simulink model "InductionHeating_bb_4"  (R2026b)
settings: Solver=FixedStepDiscrete  StopTime=0.008
PostLoadFcn:
  | Ts = 1e-6;Ts_fpga=10e-9;   R=3; Capa=300e-9;L=100e-6;Pejo_factor=1;
InitFcn:
  | Ts = 1e-6;Ts_fpga=10e-9;   R=3; Capa=300e-9;L=100e-6;Pejo_factor=1;
undefined symbols (not defined in the file or in its folder): DiscIntNeverNeededParam, ee_sli_rtmsupport, gcbh, isSetWhenUndefinedState, MATESOCwDio
libraries: fl_lib x67, nesl_utility x40, hdlsllib x32, simulink x15, eeGeneralControl x9, ee_lib x3
(part 1 of 7)
settings Model: DataTypeOverride=Off  ModifiedByFormat=sss  Creator=The MathWorks, Inc.  LastModifiedBy=sss
settings OptimizationCC: BlockReduction=off  ConditionallyExecuteInputs=off  DefaultParameterBehavior=Inlined  InheritOutputTypeSmallerThanSingle=on  ReuseModelBlockBuffer=off
settings DebuggingCC: AlgebraicLoopMsg=error  ParameterPrecisionLossMsg=none  SingleTaskRateTransMsg=error  SubsystemReferenceDiagnosticForUnitTest=warning
settings HardwareCC: ProdEndianess=Unspecified  ProdEqTarget=off  ProdHWDeviceType=ASIC/FPGA->ASIC/FPGA  ProdIntDivRoundTo=Undefined  ProdLargestAtomicFloat=None  TargetEndianess=LittleEndian  TargetHWDeviceType=Custom Processor->MATLAB Host Computer  TargetIntDivRoundTo=Zero  TargetLongLongMode=on
settings RTWCC: DLArmComputeVersion=19.05
settings SimscapeCC: SimscapeUseEnergyAccounting=off

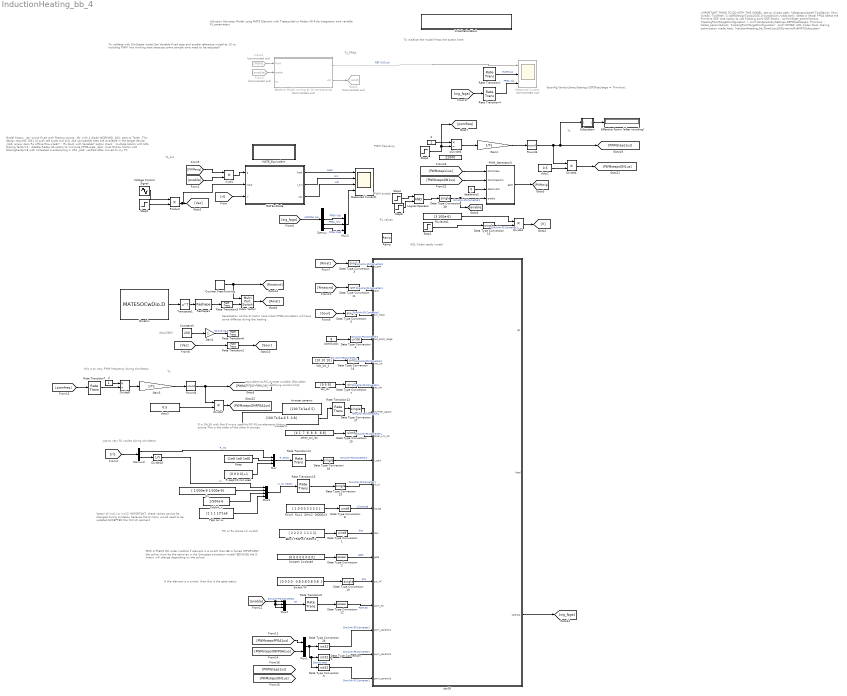
== system InductionHeating_bb_4 ==
  note: Model history
      | _aa: circuit fixed with floating source
      | _bb: with 4 diode WORKING
      | _bb1: sent to Tarek: This design requires 1041 of such cell types but only 464 compatible sites are available in the target device.
      | _bb2: erreur dans RL offline Rsw+1e6!!!
      | : RL block with VariableY option check
      | : multiple blocks with HDL sharing factor=4
      | : disable Radau IIA option to minimize FPGA area
      | _bb3: most RLCsw blocks with SharingFactor=8
      | with increased oversampling = 254
      | _bb4: verified after moved to my PC
  note: I MPORTANT THING TO DO WITH THIS MODEL:
      |
      | set-up Vivado path: hdlsetuptoolpath('ToolName','Xilinx Vivado','ToolPath','C:\AMDDesignTools\2026.1\Vivado\bin\vivado.bat');
      |
      | Select a Versal FPGA
      |
      | Select the Primitive DSP slice option to use Floating point DSP blocks.:
      | conf=hdlget_param(bdroot, 'FloatingPointTargetConfiguration' );
      | conf.VendorLibrarySettings.DSPSliceUsage= 'Primitive' ;
      | hdlset_param(bdroot, 'FloatingPointTargetConfiguration' ,conf)
      |
      | NOTES:
      | HDL Coder block sharing optimization made here: 'InductionHeating_bb_Tarek/soc16/DynamicMultMAT/Subsystem'
  note: Vdc=200V
  note: equivalent to RC inverter snubber
      | [Rsnubber Ts/Csnubber  non-rectifying current limit]
  note: D is 16x16
      | with first 8 in-out used for RC-RL-sw elements History source
      | This is the order of the other 8 sources
  note: this is to vary PWM frequency during simulation
  note: If the element is a switch, then this is the gate status
  note: just to vary RL vaules during simulation
  note: RC or RL choice (or switch)
  note: Vector of inv(L) or inv(C)
      | IMPORTANT: these values cannot be changed during simlation
      | because the D marix would need to be updated
      | EXCEPTED the first LC element
  note: IRK5 is PLECS 5th order method
      | if element is a switch then BE is forced
      | IMPORTANT: the solver must be the same as in the Simscape extraction model!
      | BECAUSE the D matrix will change depending on the solver!
  note: Ts
  note: Induction Stovetop Model using MATE Element
      | with Trapezoidal or Radau IIA Rule Integration
      | and variable RL parameters
  note: Serialisation od the D matrix here
      | Initial FPGA simulation will have some diffence during the loading
  note: HDL Coder ready model
  note: Ts
  note: Ts_FPGA
  note: To validate with SimScape model
      | Set Variable fixed step and enable reference model
      | at 10 ns including PWM
      | (not working here because some sample time need to be adjusted)
  note: Ts_1us
  note: RL values
  note: PWM frequency
  note: PWM enable
  note: fpconfig.VendorLibrarySettings.DSPSliceUsage = 'Primitive';
  note: To initialize the model
      |
      | Press the button here
  0=open 1=closed : Constant  Value=[0 0 0 0 0 0 0 0]  OutDataTypeStr=boolean  SampleTime=Ts
  1 : Constant  Value=22000  SampleTime=Ts
  3 : Constant  SampleTime=Ts
  4 : Constant  SampleTime=Ts
  BE=1 TRAP=2 IRK5=3 _ : Constant  Value="[ 2 2 2 2  1 1 1 1]"  OutDataTypeStr=single  SampleTime=Ts
  Baseline Model running at 10 nanoseconds : Subsystem  Commented=on
  Cdclink_x : Constant  Value=1/500e-6  OutDataTypeStr=single  SampleTime=Ts
  Constant : Constant  Value="[100 Ts/1e-6 5  0.8]"
  Constant3 : Constant  Value=200  SampleTime=Ts
  Counter Free-Running : hdlsllib/Sources/Counter Free-Running  NumBits=8  tsamp=-1
  Cx : Constant  Value=[ 1/300e-9 1/300e-9]  OutDataTypeStr=single  SampleTime=Ts
  Data Type Conversion{1,4,7..8,11,15..16} (7 alike) : DataTypeConversion  OutDataTypeStr=uint8  RndMeth=Nearest  SaturateOnIntegerOverflow=off
  Data Type Conversion{3,5,10,13,18..19,37..38} (8 alike) : DataTypeConversion  OutDataTypeStr=single  RndMeth=Nearest  SaturateOnIntegerOverflow=off
  Data Type Conversion12 : DataTypeConversion  OutDataTypeStr=boolean  RndMeth=Nearest  SaturateOnIntegerOverflow=off
  Data Type Conversion2 : DataTypeConversion  OutDataTypeStr=boolean  RndMeth=Nearest  SaturateOnIntegerOverflow=off
  Data Type Conversion28 : DataTypeConversion  OutDataTypeStr=int32  RndMeth=Nearest  SaturateOnIntegerOverflow=off
  Data Type Conversion6 : DataTypeConversion  OutDataTypeStr=int32  RndMeth=Nearest  SaturateOnIntegerOverflow=off
  Data Type Conversion9 : DataTypeConversion  OutDataTypeStr=int32  RndMeth=Nearest  SaturateOnIntegerOverflow=off
  Demux : Demux  Outputs=5
  Demux3 : Demux  Outputs=[1 1]
  Divide1 : Product
  Divide10 : Product  Inputs=/
  Divide4 : Product
  Divide6 : Product  Inputs=*/
  Divide7 : Product
  Divide8 : Product  Inputs=*/
  Dmatrix : Constant  Value=MATESOCwDio.D
  Effective Fpwm (after rounding) : Display
      settings: Format=bank
  From2 : From  Commented=on  GotoTag=enable
  From3 : From  Commented=on  GotoTag=PWM
  Gain1 : Gain  Gain=1/Ts
  Gain2 : Gain
  Gain3 : Gain  Gain=1/Ts
  Goto1 : Goto  Commented=on  GotoTag=vdcref
  Index Vector : MultiPortSwitch  DataPortOrder=Zero-based contiguous  Inputs=1  zeroidx=on  SaturateOnIntegerOverflow=off  InputSameDT=off
  InitializationBlock : Subsystem  AncestorBlock=simetranss/Usefulls/InitializationBlock  mask(Model Functions){InitVar=Ts = 1e-6;Ts_fpga=10e-9;   R=3; Capa=300e-9;L=100e-6;Pejo_factor=1;, InitFile=, prel=off, posl=on, inif=on}
      mask prompts: InitVar "Initialisation variables"; InitFile "Initialisation file (.m or .p)"; prel "Preload Function"; posl "PostLoad Function"; inif "InitFcn"
      mask init:
      | InitAll=[InitVar 10 InitFile];
      | if prel==1
      | 	set_param(bdroot, 'PreLoadFcn', InitAll);
      | else
      | 	set_param(bdroot, 'PreLoadFcn', '');
      | end
      | if inif==1
      | 	set_param(bdroot, 'InitFcn', InitAll);
      | else
      | 	set_param(bdroot, 'InitFcn', '');
      | end
      | 
      | if posl==1
      | 	set_param(bdroot, 'PostLoadFcn', InitAll);
      | else
      | 	set_param(bdroot, 'PostLoadFcn', '');
      | end
      | 
      | 
      | 
      | pos = get_param(gcb, 'Position');
      | width = pos(3) - pos(1); height = pos(4) - pos(2);
      mask DialogControl openfile Prompt: Open Initialisation file
      mask DialogControl openfile Callback:
      | ff1=get_param(gcb,'InitFile');
      | ff=replace(ff1,';','');
      | ff=replace(ff,'.m','');
      | ff=replace(ff,'.p','');
      | 
      | if ~isempty(strfind(ff1,'.p'))
      |     warning('p-file cannot be edited')
      | end
      | 
      | open(ff);
      mask Display:
      | text(5, height*0.5, [ ...
      |   ...
      | '- Initialisation: '  get_param(bdroot, 'InitFcn')  ...
      | ], ...
      | 'horizontalAlignment', 'left', 'verticalAlignment', 'middle') ;
  Inverter params : Constant  Value=[100 Ts/1e-6 5]
  Logical Operator : Logic  AllPortsSameDT=off  OutDataTypeStr=boolean
  MATE_Equivalent : Subsystem  mask(MATE object){MATEin='MATE', MATERT='MATERT', MATESOCvar='MATESOCwDio', subsys='InductionHeating_bb_4/MATEwDiode', discmeth=Trapezoidal, Tsx=Ts}
      mask prompts: MATEin "General MATE data structure name"; MATERT "MATE S-function parameter"; MATESOCvar "MATE-SoC output variable name"; subsys "Reference subsystem for MATE"; discmeth "Discretization"; Tsx "Sample time (s)"
      mask TypeOptions discmeth: Backward Euler | Trapezoidal |  5th order accurate fully-implicit three-stage Runge-Kutta formula (Radau IIA)
      mask DialogControl Control2 Prompt: Generate MATE equations
      mask DialogControl Control2 Callback:
      | block=gcb;
      | maskObj = Simulink.Mask.get(block); % get mask handle
      | Ts = get_param(block, 'value@Tsx'); % retrieve value for Vrated
      | sub = get_param(block, 'value@subsys'); % retrieve value for Vmin_p
      | dd = get_param(block, 'value@discmeth'); % retrieve value for Vmin_p
      | mm = get_param(block, 'value@MATEin'); % retrieve value for Vmin_p
      | mrt = get_param(block, 'value@MATERT'); % retrieve value for Vmin_p
      | msoc = get_param(block, 'value@MATESOCvar'); % retrieve value for Vmin_p
      | if dd==3
      |     dd=5;
      | end
      | %Tss=get_param(block,'Ts')
      | [MATEx, MATERTx]= MakeMate2(sub , dd, Ts);
      | %MATEin='MATE';
      | assignin("base",mm,MATEx);
      | assignin("base",mrt,MATERTx);
      | [MATESOCx]=MateConvertForFPGA(MATEx,2);  % don;t forget option 2
      | assignin("base",msoc,MATESOCx);
  MATEwDiode : Subsystem
  Measured Current : Scope  Commented=on  NumInputPorts=3
      settings: ActiveDisplayYMinimum=-142.71321105957031  ActiveDisplayYMaximum=758.74385070800781
  Measured Current1 : Scope  NumInputPorts=4
      settings: ActiveDisplayYMinimum=-62.985793783247914  ActiveDisplayYMaximum=66.216303930478091
  Mux : Mux  Inputs=3
  Mux1 : Mux  Inputs=2
  Mux2 : Mux  Inputs=3
  Mux3 : Mux  Inputs=3
  Mux5 : Mux
  PWM_Generator3 : Subsystem
      mask Display: disp(' PWM \n Generator ')
  Pejo sw Lx : Constant  Value=[1 1 1 1]*1e6  OutDataTypeStr=single  SampleTime=Ts
  Product : Product
  R pejo=0 not used : Constant  Value=[0 0 0 0]+1  OutDataTypeStr=single  SampleTime=Ts
  RC=0  RL=1  SW=2  DIODE=3 : Constant  Value=[ 1 0 0 0 3 3 3 3 ]  OutDataTypeStr=single  SampleTime=Ts
  RLvlaues1 : Constant  Value=[3 100e-6]  OutDataTypeStr=single  SampleTime=Ts
  Ramp : simulink/Sources/Ramp  slope=-0.1*1000  start=0.004  InitialOutput=1
  Rate Transition1 : RateTransition  Integrity=off
  Rate Transition{5,7,13..15} (5 alike) : RateTransition  Integrity=off  OutPortSampleTime=Ts
  Rate Transition2 : RateTransition  OutPortSampleTime=1e-06
  Rate Transition3 : RateTransition  OutPortSampleTime=1e-06
  Rate Transition4 : RateTransition  Integrity=off
  Rate Transition6 : RateTransition  OutPortSampleTime=1e-06
  Rcap : Constant  Value=[1e8 1e8 1e8]  OutDataTypeStr=single  SampleTime=Ts
  Reshape1 : Reshape
  Round3 : Rounding  Operator=round
  Round4 : Rounding  Operator=round
  Step1 : Step  Time=0.004  InitialValue=1  FinalValue=0.9  SampleTime=Ts
  Step2 : Step  Time=0.002  SampleTime=Ts
  Step3 : Step  Time=0.001  SampleTime=Ts
  Step4 : Step  Time=0.003  InitialValue=25000  FinalValue=22000  SampleTime=Ts
  Step6 : Step  Time=0.005  InitialValue=1  FinalValue=0  SampleTime=Ts
  Subsystem : Subsystem
  Switch VF : Constant  Value="[0 0 0 0   0.8 0.8 0.8 0.8  ]"  OutDataTypeStr=single  SampleTime=Ts
  Transpose1 : Math  Operator=transpose
  UserOutidx : Constant  Value=9  SampleTime=Ts
  Vdc_idx_1 : Constant  Value=[10 10 10]  SampleTime=Ts
  Voltage Control Signal : Sin  Amplitude=220  Frequency=500 * 2 *pi  SampleTime=Ts
  deadtime2 : Constant  Value=0  SampleTime=Ts
  duty2 : Constant  Value=0.5  SampleTime=Ts
  duty3 : Constant  Value=0.5  SampleTime=Ts
  iac_idx : Constant  Value=[9 9 9]  SampleTime=Ts
  mult1 : Product
  other_src_idx : Constant  Value="[4 1  7  8  8  8   8 8]"  SampleTime=Ts
  soc16 : Subsystem  TreatAsAtomicUnit=on
  wires:
  Rate Transition1/1 -> Measured Current/2  "MATE 1us"
  Baseline Model running at 10 nanoseconds/1(i) -> Measured Current/1  "REF (0.01 us)"
  From2/1 -> Baseline Model running at 10 nanoseconds/2(enable)
  Baseline Model running at 10 nanoseconds/2(vdc) -> Goto1/1
  From3/1 -> Baseline Model running at 10 nanoseconds/1(PWM)
  Rate Transition4/1 -> Measured Current/3  "FPGA 1us"
  [Rmat] -> Data Type Conversion3/1
  Counter Free-Running/1 -> Index Vector/1, [Rmatcnt]
  Dmatrix/1 -> Transpose1/1
  Transpose1/1 -> Reshape1/1
  Reshape1/1 -> Rate Transition3/1
  Rate Transition3/1 -> Index Vector/2
  Gain2/1 -> Rate Transition6/1  "Source input"
  [Rmatcnt] -> Data Type Conversion11/1
  Index Vector/1 -> [Rmat]
  [Sour] -> Data Type Conversion5/1
  Constant3/1 -> Gain2/1
  [PWMstepsFPGA1us] -> Mux1/1
  [PWMstepsONFPGA1us] -> Mux1/2
  Mux1/1 -> Data Type Conversion9/1, Data Type Conversion6/1, Data Type Conversion28/1  "Source input"
  Data Type Conversion28/1 -> soc16/16(pwm_params1)  "Simulink-PS Converter1"
  Data Type Conversion37/1 -> soc16/7(inverter_param)  "Simulink-PS Converter1"
  [PWMstepsON1us] -> PWM_Generator3/2(PWMstepsON)
  [PWMsteps1us] -> PWM_Generator3/1(PWMsteps)
  deadtime2/1 -> PWM_Generator3/3(deatime(s))
  duty2/1 -> Divide4/2
  Divide4/1 -> [PWMstepsON1us]
  Round3/1 -> Divide4/1, Subsystem/1(In1), [PWMsteps1us]
  Divide6/1 -> Gain1/1
  Gain1/1 -> Round3/1
  3/1 -> Divide6/1
  Data Type Conversion38/1 -> [enable], PWM_Generator3/4(enable)  "Simulink-PS Converter1"
  PWM_Generator3/1(gate) -> [PWMavg]
  Data Type Conversion3/1 -> soc16/1(d_port)  "Simulink-PS Converter1"
  Data Type Conversion11/1 -> soc16/2(dcnt)  "Simulink-PS Converter1"
  Data Type Conversion5/1 -> soc16/3(src_input)  "Simulink-PS Converter1"
  4/1 -> Divide8/1
  Divide8/1 -> Gain3/1
  Gain3/1 -> Round4/1
  duty3/1 -> Divide7/2
  Rate Transition7/1 -> Divide8/2
  Round4/1 -> [PWMstepsFPGA1us], Divide7/1
  Divide7/1 -> [PWMstepsONFPGA1us]
  Rate Transition13/1 -> Data Type Conversion37/1
  [sig_fpga] -> Rate Transition4/1
  [pwmfreq] -> Rate Transition7/1
  other_src_idx/1 -> Data Type Conversion15/1
  iac_idx/1 -> Data Type Conversion7/1
  UserOutidx/1 -> Data Type Conversion4/1
  Data Type Conversion4/1 -> soc16/4(out_start_range)  "Simulink-PS Converter1"
  Vdc_idx_1/1 -> Data Type Conversion16/1  "Simulink-PSConverter1"
  Data Type Conversion7/1 -> soc16/6(iac_idx)  "Simulink-PS Converter1"
  Data Type Conversion16/1 -> soc16/5(vdc_idx)  "Simulink-PS Converter1"
  Data Type Conversion15/1 -> soc16/8(other_src_idx)  "Simulink-PS Converter1"
  Mux5/1 -> Rate Transition15/1  "Lx_Cx vector"
  Demux3/2 -> Divide10/1
  Mux/1 -> Rate Transition14/1  "R vector"
  Data Type Conversion18/1 -> soc16/9(r_port)  "Simulink-PS Converter1"
  Data Type Conversion19/1 -> soc16/10(lx_cx)  "Simulink-PS Converter1"
  Rate Transition14/1 -> Data Type Conversion18/1
  Rate Transition15/1 -> Data Type Conversion19/1
  Data Type Conversion8/1 -> soc16/11(lctype)  "LCswtype"
  Data Type Conversion1/1 -> soc16/12(disc)  "disc"
  Data Type Conversion2/1 -> soc16/13(gate)  "gate"
  RC=0  RL=1  SW=2  DIODE=3/1 -> Data Type Conversion8/1
  0=open 1=closed/1 -> Data Type Conversion2/1
  BE=1 TRAP=2 IRK5=3 _/1 -> Data Type Conversion1/1
  Rate Transition5/1 -> Data Type Conversion12/1
  Data Type Conversion12/1 -> soc16/15(pwm_en)  "PWM en"
  Data Type Conversion6/1 -> soc16/17(pwm_params2)  "Simulink-PS Converter1"
  Data Type Conversion9/1 -> soc16/18(pwm_params3)  "Simulink-PS Converter1"
  [enable] -> Mux2/3, Mux2/2, Mux2/1  "Simulink-PS Converter1"
  Mux2/1 -> Rate Transition5/1  "en"
  mult1/1 -> MATEwDiode/1(g)
  [PWMavg] -> mult1/1
  [enable] -> mult1/2
  MATEwDiode/3(vdc) -> Measured Current1/3  "Vdc"
  MATEwDiode/1(iload) -> Measured Current1/1  "Iload"
  MATEwDiode/2(i_src) -> Measured Current1/2  "Isrc"
  Subsystem/1(Out1) -> Effective Fpwm (after rounding)/1
  Switch VF/1 -> Data Type Conversion10/1
  Data Type Conversion10/1 -> soc16/14(sw_VF)  "disc"
  Step4/1 -> [pwmfreq], Divide6/2
  [Vac] -> Rate Transition2/1
  Rate Transition2/1 -> [Sour]
  Demux3/1 -> Mux/1  "R_ind"
  Rcap/1 -> Mux/2
  R pejo=0 not used/1 -> Mux/3
  Divide10/1 -> Mux5/1  "Lx"
  Cx/1 -> Mux5/2
  Cdclink_x/1 -> Mux5/3
  Pejo sw Lx/1 -> Mux5/4
  soc16/3(userout) -> [sig_fpga]
  Divide1/1 -> [rl]
  Data Type Conversion13/1 -> Divide1/2  "Simulink-PS Converter1"
  RLvlaues1/1 -> Divide1/1
  [rl] -> MATEwDiode/3(rl)
  [rl] -> Demux3/1
  Step2/1 -> Logical Operator/1
  Step6/1 -> Logical Operator/2
  Logical Operator/1 -> Data Type Conversion38/1
  Step3/1 -> Product/2
  Voltage Control Signal/1 -> Product/1
  Product/1 -> MATEwDiode/2(Input), [Vac]
  Constant/1 -> Rate Transition13/1
  [sig_fpga] -> Demux/1  "vdcFPGA 1us"
  Demux/5 -> Mux3/3  "FPGA Iload"
  Mux3/1 -> Measured Current1/4
  Demux/4 -> Mux3/2  "FPGA_Isrc"
  Demux/3 -> Mux3/1  "FPGA Vdc"
  Step1/1 -> Data Type Conversion13/1

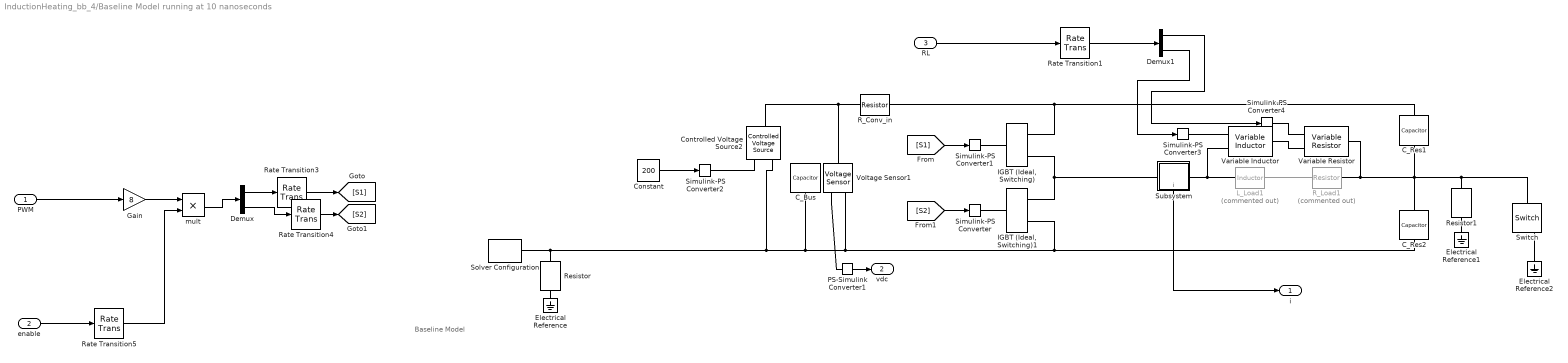
== system InductionHeating_bb_4/Baseline Model running at 10 nanoseconds ==
  note: Baseline Model
  PWM : Inport
  enable : Inport  Port=2
  RL : Inport  Port=3
  C_Bus : fl_lib/Electrical/Electrical Elements/Capacitor  c=5e-5 F  r=0 Ohm  g=0 1/Ohm  i_specify=off  i_priority=None  i=0 A  i_nominal_specify=off  i_nominal_value=1  i_nominal_unit=A  v_specify=off  v_priority=None  v=0 V  v_nominal_specify=off  v_nominal_value=1  v_nominal_unit=V  vc_specify=off  vc_priority=High  vc=0 V  vc_nominal_specify=off  vc_nominal_value=1  vc_nominal_unit=V
      settings: AttributesFormatString=%<c> %<c_unit>
  C_Res1 : fl_lib/Electrical/Electrical Elements/Capacitor  c=300e-9 F  r=0 Ohm  g=0 1/Ohm  i_specify=off  i_priority=None  i=0 A  i_nominal_specify=off  i_nominal_value=1  i_nominal_unit=A  v_specify=off  v_priority=None  v=0 V  v_nominal_specify=off  v_nominal_value=1  v_nominal_unit=V  vc_specify=off  vc_priority=High  vc=0 V  vc_nominal_specify=off  vc_nominal_value=1  vc_nominal_unit=V
      settings: AttributesFormatString=%<c> %<c_unit>
  C_Res2 : fl_lib/Electrical/Electrical Elements/Capacitor  c=300e-9 F  r=0 Ohm  g=0 1/Ohm  i_specify=off  i_priority=None  i=0 A  i_nominal_specify=off  i_nominal_value=1  i_nominal_unit=A  v_specify=off  v_priority=None  v=0 V  v_nominal_specify=off  v_nominal_value=1  v_nominal_unit=V  vc_specify=off  vc_priority=High  vc=0 V  vc_nominal_specify=off  vc_nominal_value=1  vc_nominal_unit=V
      settings: AttributesFormatString=%<c> %<c_unit>
  Constant : Constant  Value=200
  Controlled Voltage Source2 : fl_lib/Electrical/Electrical Sources/Controlled Voltage Source
  Demux : Demux  Outputs=2
  Demux1 : Demux  Outputs=2
  Electrical Reference : fl_lib/Electrical/Electrical Elements/Electrical Reference
  Electrical Reference1 : fl_lib/Electrical/Electrical Elements/Electrical Reference
  Electrical Reference2 : fl_lib/Electrical/Electrical Elements/Electrical Reference
  Gain : Gain  Gain=8
  "IGBT (Ideal, Switching)" : ee_lib/Semiconductors & Converters/IGBT (Ideal, Switching)  port_option=ee.enum.controlport.ps  Vf=0.8 V  Ron=0.001 Ohm  Goff=1e-8 1/Ohm  Vth=6 V  diode_param=2  diode_Vf=0.8 V  diode_Ron=0.001 Ohm  diode_Goff=1e-8 1/Ohm  diode_C=50e-9 F  diode_iRM=-235 A  diode_iF=300 A  diode_idot=-50 A/us  diode_trr_param=1  diode_trr_factor=3  diode_trr=15 us  diode_Qrr=1500 s*uA  ice_specify=off  ice_priority=None  ice=0 A  ice_nominal_specify=off  ice_nominal_value=1  ice_nominal_unit=A  vce_specify=off  vce_priority=None  vce=0 V  vce_nominal_specify=off  vce_nominal_value=1  vce_nominal_unit=V  vge_specify=off  vge_priority=None  vge=0 V  vge_nominal_specify=off  vge_nominal_value=1  vge_nominal_unit=V  thermal_loss_option=ee.enum.converters.thermalLossOption.constantvalues  Von_data=[0, .1, .6, .8, 1, 1.3, 1.6, 2, 2.4; 0, .1, .7, 1, 1.2, 1.5, 1.9, 2.4, 2.8] V  Tj=[298.15, 398.15] K  Iout_data=[0, .1, 1, 5, 10, 20, 40, 70, 100] A  Eon_data=[0, .0024, .024, .12, .2, .48, 1.04, 2.16, 3.24; 0, .003, .03, .15, .25, .6, 1.3, 2.7, 4.05] * 1e-3 J  Eoff_data=[0, .0007, .0066, .033, .066, .17, .33, .83, 1.5; 0, .001, .01, .05, .1, .25, .5, 1.2, 2.2] * 1e-3 J  Eon_data_3D=[zeros(2, 9, 3)] J  Eoff_data_3D=[zeros(2, 9, 3)] J  Tj_loss=[298.15, 398.15] K  Iout_data_loss=[0, .1, 1, 5, 10, 20, 40, 70, 100] A  tabulateWithVce=false  Vce_loss=[0, 150, 300] V  Eon_scalar=22.86e-3 J  Eoff_scalar=17.14e-3 J  Voff=300 V  Iout_scalar=600 A  useCurrentFromPreviousCycle=false  useVoltageFromPreviousCycle=false  diodeModelType=ee.enum.converters.diodeModelType.pwl  diodeTableType=ee.enum.diode.tableType.IfMat  diode_ReverseIVType=ee.enum.diode.diodeReverseIV.constant  diode_IfMat=[.07, .12, .19, 1.75, 4.24, 7.32, 11.2; .16, .3, .72, 2.14, 4.02, 6.35, 9.12] A  diode_VfMat=[.9, 1.15, 1.25, 1.5, 1.75, 2.17, 2.6, 2.85; .58, .68, .75, 1.1, 1.38, 1.77, 2.27, 2.7] V  diode_TjVec=[25, 125] degC  diode_VfVec=[.5, .7, .9, 1.3, 1.7, 2.1, 2.5] V  diode_IfVec=[.1, .2, .5, 1, 2, 4, 7, 10] A  diode_IrMat=[1e-06, 2e-06, 5e-06, 1e-05, 2.5e-05, 5e-05, .0001; 2e-06, 5e-06, 1e-05, 4e-05, 8e-05, .0002, .0005] A  diode_VrMat=[10, 100, 200, 250, 300, 325, 350; 10, 70, 160, 220, 270, 300, 320] V  diode_VrVec=[10, 20, 40, 50, 70, 80, 100] V  diode_IrVec=[1e-06, 2e-06, 5e-06, 1e-05, 2e-05, 5e-05, .0001] A  diode_Vr=-600 V  diode_Ls=150 nH  diode_Erec=0.03 J  diode_rec_loss_model=ee.enum.diode.reverseRecoveryModel.fixed  diode_ErecVal=0 J  diode_scaleWithIandV=true  diode_ErecMat=zeros(2, 3) J  diode_TjrecVec=[298.15, 398.15] K  diode_IfrecVec=[.1, 1, 10] A  diode_IrecVal=10 A  diode_VrecVal=10 V  diode_tFilter=1 / 1000 / 100 s  separateThermalPortForDiode=false  thermal_network_parameterization=ee.enum.thermalNetworkTopology.external  Rth=[.08, .5] K/W  Rth_Cauer=[.08, .1, .5] K/W  Rth_Foster=[.08, .14, .22, .16] K/W  thermal_mass_parameterization=ee.enum.thermalNetwork.timeconstant  thermal_mass=[.01, .5] J/K  thermal_mass_Cauer=[.01, .1, .5] J/K  thermal_mass_Foster=[.001, .005, .05, .5] J/K  thermal_time_constant=[.001, .2] s  thermal_time_constant_Cauer=[.001, .1, .2] s  thermal_time_constant_Foster=[7e-05, .0007, .01, .08] s  thermal_mass_initial_temperatures=[25, 25] degC  thermal_mass_initial_temperatures_Cauer=[25, 25, 25] degC  junction_thermal_mass=0.01 J/K  Tvec_initial_Foster=[25, 25, 25, 25] degC  RthDiode=[.03, .2] K/W  RthCauerDiode=[.03, .1, .2] K/W  RthFosterDiode=[.03, .2] K/W  thermalMassDiode=[3, 25] J/K  thermalMassCauerDiode=[3, 10, 25] J/K  thermalMassFosterDiode=[33, 50] J/K  thermalTauDiode=[.1, 5] s  thermalTauCauerDiode=[.1, 1, 5] s  thermalTauFosterDiode=[1, 10] s  thermalMassInitTempDiode=[25, 25] degC  thermalMassInitTempCauerDiode=[25, 25, 25] degC  junctionthermalMassDiode=0.1 J/K  TVecInitialFosterDiode=[25, 25, 25, 25] degC  no_thermal_network=0  IGBT_junction_temperature_specify=off  IGBT_junction_temperature_priority=None  IGBT_junction_temperature=25 degC  IGBT_junction_temperature_nominal_specify=off  IGBT_junction_temperature_nominal_value=1  IGBT_junction_temperature_nominal_unit=degC  diode_junction_temperature_specify=off  diode_junction_temperature_priority=None  diode_junction_temperature=25 degC  diode_junction_temperature_nominal_specify=off  diode_junction_temperature_nominal_value=1  diode_junction_temperature_nominal_unit=degC  Qj_specify=off  Qj_priority=None  Qj=0 W  Qj_nominal_specify=off  Qj_nominal_value=1  Qj_nominal_unit=W  accumulatedSwitchingLosses_specify=off  accumulatedSwitchingLosses_priority=None  accumulatedSwitchingLosses=0 J
  "IGBT (Ideal, Switching)1" : ee_lib/Semiconductors & Converters/IGBT (Ideal, Switching)  port_option=ee.enum.controlport.ps  Vf=0.8 V  Ron=0.001 Ohm  Goff=1e-8 1/Ohm  Vth=6 V  diode_param=2  diode_Vf=0.8 V  diode_Ron=0.001 Ohm  diode_Goff=1e-8 1/Ohm  diode_C=50e-9 F  diode_iRM=-235 A  diode_iF=300 A  diode_idot=-50 A/us  diode_trr_param=1  diode_trr_factor=3  diode_trr=15 us  diode_Qrr=1500 s*uA  ice_specify=off  ice_priority=None  ice=0 A  ice_nominal_specify=off  ice_nominal_value=1  ice_nominal_unit=A  vce_specify=off  vce_priority=None  vce=0 V  vce_nominal_specify=off  vce_nominal_value=1  vce_nominal_unit=V  vge_specify=off  vge_priority=None  vge=0 V  vge_nominal_specify=off  vge_nominal_value=1  vge_nominal_unit=V  thermal_loss_option=ee.enum.converters.thermalLossOption.constantvalues  Von_data=[0, .1, .6, .8, 1, 1.3, 1.6, 2, 2.4; 0, .1, .7, 1, 1.2, 1.5, 1.9, 2.4, 2.8] V  Tj=[298.15, 398.15] K  Iout_data=[0, .1, 1, 5, 10, 20, 40, 70, 100] A  Eon_data=[0, .0024, .024, .12, .2, .48, 1.04, 2.16, 3.24; 0, .003, .03, .15, .25, .6, 1.3, 2.7, 4.05] * 1e-3 J  Eoff_data=[0, .0007, .0066, .033, .066, .17, .33, .83, 1.5; 0, .001, .01, .05, .1, .25, .5, 1.2, 2.2] * 1e-3 J  Eon_data_3D=[zeros(2, 9, 3)] J  Eoff_data_3D=[zeros(2, 9, 3)] J  Tj_loss=[298.15, 398.15] K  Iout_data_loss=[0, .1, 1, 5, 10, 20, 40, 70, 100] A  tabulateWithVce=false  Vce_loss=[0, 150, 300] V  Eon_scalar=22.86e-3 J  Eoff_scalar=17.14e-3 J  Voff=300 V  Iout_scalar=600 A  useCurrentFromPreviousCycle=false  useVoltageFromPreviousCycle=false  diodeModelType=ee.enum.converters.diodeModelType.pwl  diodeTableType=ee.enum.diode.tableType.IfMat  diode_ReverseIVType=ee.enum.diode.diodeReverseIV.constant  diode_IfMat=[.07, .12, .19, 1.75, 4.24, 7.32, 11.2; .16, .3, .72, 2.14, 4.02, 6.35, 9.12] A  diode_VfMat=[.9, 1.15, 1.25, 1.5, 1.75, 2.17, 2.6, 2.85; .58, .68, .75, 1.1, 1.38, 1.77, 2.27, 2.7] V  diode_TjVec=[25, 125] degC  diode_VfVec=[.5, .7, .9, 1.3, 1.7, 2.1, 2.5] V  diode_IfVec=[.1, .2, .5, 1, 2, 4, 7, 10] A  diode_IrMat=[1e-06, 2e-06, 5e-06, 1e-05, 2.5e-05, 5e-05, .0001; 2e-06, 5e-06, 1e-05, 4e-05, 8e-05, .0002, .0005] A  diode_VrMat=[10, 100, 200, 250, 300, 325, 350; 10, 70, 160, 220, 270, 300, 320] V  diode_VrVec=[10, 20, 40, 50, 70, 80, 100] V  diode_IrVec=[1e-06, 2e-06, 5e-06, 1e-05, 2e-05, 5e-05, .0001] A  diode_Vr=-600 V  diode_Ls=150 nH  diode_Erec=0.03 J  diode_rec_loss_model=ee.enum.diode.reverseRecoveryModel.fixed  diode_ErecVal=0 J  diode_scaleWithIandV=true  diode_ErecMat=zeros(2, 3) J  diode_TjrecVec=[298.15, 398.15] K  diode_IfrecVec=[.1, 1, 10] A  diode_IrecVal=10 A  diode_VrecVal=10 V  diode_tFilter=1 / 1000 / 100 s  separateThermalPortForDiode=false  thermal_network_parameterization=ee.enum.thermalNetworkTopology.external  Rth=[.08, .5] K/W  Rth_Cauer=[.08, .1, .5] K/W  Rth_Foster=[.08, .14, .22, .16] K/W  thermal_mass_parameterization=ee.enum.thermalNetwork.timeconstant  thermal_mass=[.01, .5] J/K  thermal_mass_Cauer=[.01, .1, .5] J/K  thermal_mass_Foster=[.001, .005, .05, .5] J/K  thermal_time_constant=[.001, .2] s  thermal_time_constant_Cauer=[.001, .1, .2] s  thermal_time_constant_Foster=[7e-05, .0007, .01, .08] s  thermal_mass_initial_temperatures=[25, 25] degC  thermal_mass_initial_temperatures_Cauer=[25, 25, 25] degC  junction_thermal_mass=0.01 J/K  Tvec_initial_Foster=[25, 25, 25, 25] degC  RthDiode=[.03, .2] K/W  RthCauerDiode=[.03, .1, .2] K/W  RthFosterDiode=[.03, .2] K/W  thermalMassDiode=[3, 25] J/K  thermalMassCauerDiode=[3, 10, 25] J/K  thermalMassFosterDiode=[33, 50] J/K  thermalTauDiode=[.1, 5] s  thermalTauCauerDiode=[.1, 1, 5] s  thermalTauFosterDiode=[1, 10] s  thermalMassInitTempDiode=[25, 25] degC  thermalMassInitTempCauerDiode=[25, 25, 25] degC  junctionthermalMassDiode=0.1 J/K  TVecInitialFosterDiode=[25, 25, 25, 25] degC  no_thermal_network=0  IGBT_junction_temperature_specify=off  IGBT_junction_temperature_priority=None  IGBT_junction_temperature=25 degC  IGBT_junction_temperature_nominal_specify=off  IGBT_junction_temperature_nominal_value=1  IGBT_junction_temperature_nominal_unit=degC  diode_junction_temperature_specify=off  diode_junction_temperature_priority=None  diode_junction_temperature=25 degC  diode_junction_temperature_nominal_specify=off  diode_junction_temperature_nominal_value=1  diode_junction_temperature_nominal_unit=degC  Qj_specify=off  Qj_priority=None  Qj=0 W  Qj_nominal_specify=off  Qj_nominal_value=1  Qj_nominal_unit=W  accumulatedSwitchingLosses_specify=off  accumulatedSwitchingLosses_priority=None  accumulatedSwitchingLosses=0 J
  L_Load1 : fl_lib/Electrical/Electrical Elements/Inductor  Commented=on  l=100e-6 H  r=0 Ohm  g=1e-12 1/Ohm  i_specify=off  i_priority=None  i=0 A  i_nominal_specify=off  i_nominal_value=1  i_nominal_unit=A  v_specify=off  v_priority=None  v=0 V  v_nominal_specify=off  v_nominal_value=1  v_nominal_unit=V  i_L_specify=off  i_L_priority=High  i_L=0 A  i_L_nominal_specify=off  i_L_nominal_value=1  i_L_nominal_unit=A
      settings: AttributesFormatString=%<l> %<l_unit>
  PS-Simulink Converter1 : nesl_utility/PS-Simulink Converter  PhysicalDomain=network_engine_domain  SubClassName=ps_output  LeftPortType=input  RightPortType=output  PseudoPeriodic=off  Frequencies=[]  VectorFormat=1-D array  Unit=inherit  AffineConversion=off
  R_Conv_in : fl_lib/Electrical/Electrical Elements/Resistor  R=0.01 Ohm  i_specify=off  i_priority=None  i=0 A  i_nominal_specify=off  i_nominal_value=1  i_nominal_unit=A  v_specify=off  v_priority=None  v=0 V  v_nominal_specify=off  v_nominal_value=1  v_nominal_unit=V
      settings: AttributesFormatString=%<R> %<R_unit>
  R_Load1 : fl_lib/Electrical/Electrical Elements/Resistor  Commented=on  R=3 Ohm  i_specify=off  i_priority=None  i=0 A  i_nominal_specify=off  i_nominal_value=1  i_nominal_unit=A  v_specify=off  v_priority=None  v=0 V  v_nominal_specify=off  v_nominal_value=1  v_nominal_unit=V
      settings: AttributesFormatString=%<R> %<R_unit>
  Rate Transition{1,3..5} (4 alike) : RateTransition
  Resistor : fl_lib/Electrical/Electrical Elements/Resistor  R=1000000 Ohm  i_specify=off  i_priority=None  i=0 A  i_nominal_specify=off  i_nominal_value=1  i_nominal_unit=A  v_specify=off  v_priority=None  v=0 V  v_nominal_specify=off  v_nominal_value=1  v_nominal_unit=V
  Resistor1 : fl_lib/Electrical/Electrical Elements/Resistor  R=1e8 Ohm  i_specify=off  i_priority=None  i=0 A  i_nominal_specify=off  i_nominal_value=1  i_nominal_unit=A  v_specify=off  v_priority=None  v=0 V  v_nominal_specify=off  v_nominal_value=1  v_nominal_unit=V
  Simulink-PS Converter{,1..4} (5 alike) : nesl_utility/Simulink-PS Converter  PhysicalDomain=network_engine_domain  SubClassName=ps_input  LeftPortType=input  RightPortType=output  PseudoPeriodic=off  Frequencies=[]  NoiseDistribution=none  NoiseParameters=[]  Unit=1  AffineConversion=off  FilteringAndDerivatives=provide  SimscapeFilterOrder=1  InputFilterTimeConstant=0.001  UdotUserProvided=0
  Solver Configuration : nesl_utility/Solver Configuration  PhysicalDomain=network_engine_domain  SubClassName=solver  LeftPortType=input  RightPortType=generic  Tones=[]  Harmonics=[]  SimulateNoise=off  Profile=off  UseLocalSampling=off  EnableSwitchedLinearOptims=on  FrequencyDomain=off  UseCCode=off  RelTol=0.001  AbsTol=1e-06  MinStep=1e-09  ToWorkspace=off  RevertToSquareIcSolve=off  NumHomotopyIterations=100  PhasorMode=off  PhasorModeNumHarmonics=1  ConsistencySolver=NEWTON_FTOL  IndexReductionMethod=DerivativeReplacement  DoDC=off  ResidualTolerance=1e-09  ConsistencyTolSource=GLOBAL  ConsistencyAbsTol=0.001  ConsistencyRelTol=0.001  ConsistencyTolFactor=0.001  UseLocalSolver=off  LocalSolverChoice=NE_TRAPEZOIDAL_ADVANCER  ResolveIndetEquations=on  FunctionEvalNumThread=1  LocalSolverSampleTime=1e-6  DoFixedCost=off  MaxNonlinIter=3  MaxModeIter=2  ComputeImpulses=off  ImpulseIterations=2  LinearAlgebra=auto  LinearAlgebraNumThread=0  EquationFormulation=NE_TIME_EF  DelaysMemoryBudget=1024  AutomaticFiltering=on  FilteringTimeConstant=0.001  PartitionStorageMethod=AS_NEEDED  PartitionMemoryBudget=1024  PartitionMethod=ROBUST  MultibodyUseLocalSolver=off  MultibodyLocalSolverChoice=ODE1  MultibodyLocalSolverSampleTime=0.001
  Subsystem : Subsystem
      settings: PortSchema="{\"entries\":[{\"content\":{\"sides\":[{\"content\":{\"connectorIds\":[\"LConn1\"]},\"type\":\"ConnectorPlacement.EquallySpacedRectSide\",\"uuid\":\"076679af-cf2d-42cc-92f3-c0233f61b32a\"},{\"content\":{\"connectorIds\":[\"RConn1\"],\"side\":\"RIGHT\"},\"type\":\"ConnectorPlacement.EquallySpacedRectSide\",\"uuid\":\"b256d27d-4c49-40e6-9ef5-c4a9651a2296\"},{\"content\":{\"connectorIds\":[],\"side\":\"TOP\"},\"type\":\"ConnectorPlacement.EquallySpacedRectSide\",\"uuid\":\"7c2293c3-6569-452f-b68e-58f8d8f046a0\"},{\"content\":{\"connectorIds\":[\"Out1\"],\"side\":\"BOTTOM\"},\"type\":\"ConnectorPlacement.EquallySpacedRectSide\",\"uuid\":\"0b29af64-854a-4551-84ea-ae8713af1006\"}]},\"type\":\"ConnectorPlacement.EquallySpacedConnector\",\"uuid\":\"813ba93f-15bf-4e08-b2ea-5f69cefe7eb7\"}],\"packageUris\":[\"http://schema.mathworks.com/mf0/Connector/R2020b\"],\"version\":\"1.0\"}"
  Switch : fl_lib/Electrical/Electrical Elements/Switch  R_closed=0.01 Ohm  G_open=1e-9 1/Ohm  Threshold=0.5  i_specify=off  i_priority=None  i=0 A  i_nominal_specify=off  i_nominal_value=1  i_nominal_unit=A  v_specify=off  v_priority=None  v=0 V  v_nominal_specify=off  v_nominal_value=1  v_nominal_unit=V
  Variable Inductor : ee_lib/Passive/Variable Inductor  prm=2  Lmin=1e-6 H  g=1e-9 1/Ohm  i0=0 A  phi0=0 Wb
      settings: InternalSimscapePortConfiguration="{\"Bottom\":[],\"Left\":[{\"id\":\"L\",\"label\":\"L\",\"type\":\"input\"},{\"id\":\"p\",\"label\":\"+\",\"type\":\"foundation.electrical.electrical\"}],\"Right\":[{\"id\":\"n\",\"label\":\"-\",\"type\":\"foundation.electrical.electrical\"}],\"Top\":[]}"
  Variable Resistor : fl_lib/Electrical/Electrical Elements/Variable Resistor  Rmin=1e-9 Ohm  thermalEnable=false  thermal_mass=1 J/K  i_specify=off  i_priority=None  i=0 A  i_nominal_specify=off  i_nominal_value=1  i_nominal_unit=A  v_specify=off  v_priority=None  v=0 V  v_nominal_specify=off  v_nominal_value=1  v_nominal_unit=V  T_specify=off  T_priority=None  T=300 K  T_nominal_specify=off  T_nominal_value=1  T_nominal_unit=K
  Voltage Sensor1 : fl_lib/Electrical/Electrical Sensors/Voltage Sensor
  mult : Product
  i : Outport
  vdc : Outport  Port=2
  wires:
  [S2] -> Simulink-PS Converter/1
  [S1] -> Simulink-PS Converter1/1
  Subsystem/1(i) -> i/1
  Demux/1 -> Rate Transition3/1
  Demux/2 -> Rate Transition4/1
  PWM/1 -> Gain/1
  Rate Transition3/1 -> [S1]
  Rate Transition4/1 -> [S2]
  mult/1 -> Demux/1
  Gain/1 -> mult/1
  enable/1 -> Rate Transition5/1
  Rate Transition5/1 -> mult/2
  PS-Simulink Converter1/1 -> vdc/1
  Constant/1 -> Simulink-PS Converter2/1
  RL/1 -> Rate Transition1/1
  Demux1/1 -> Simulink-PS Converter4/1
  Demux1/2 -> Simulink-PS Converter3/1
  Rate Transition1/1 -> Demux1/1
  connections:
  Electrical Reference/LConn1 -- Resistor/RConn1
  Resistor1/LConn1 -- Variable Resistor/RConn1 -- R_Load1/RConn1 -- C_Res2/LConn1 -- C_Res1/RConn1 -- Switch/LConn1
  C_Res1/LConn1 -- "IGBT (Ideal, Switching)"/RConn1 -- R_Conv_in/RConn1
  Simulink-PS Converter/RConn1 -- "IGBT (Ideal, Switching)1"/LConn1
  Resistor/LConn1 -- Controlled Voltage Source2/RConn2 -- C_Res2/RConn1 -- "IGBT (Ideal, Switching)1"/RConn2 -- Voltage Sensor1/RConn2 -- C_Bus/RConn1 -- Solver Configuration/RConn1
  Subsystem/LConn1 -- "IGBT (Ideal, Switching)"/RConn2 -- "IGBT (Ideal, Switching)1"/RConn1
  Voltage Sensor1/LConn1 -- R_Conv_in/LConn1 -- Controlled Voltage Source2/LConn1
  Subsystem/RConn1 -- Variable Inductor/LConn2 -- L_Load1/LConn1
  L_Load1/RConn1 -- R_Load1/LConn1
  Simulink-PS Converter1/RConn1 -- "IGBT (Ideal, Switching)"/LConn1
  Voltage Sensor1/RConn1 -- PS-Simulink Converter1/LConn1
  Controlled Voltage Source2/RConn1 -- Simulink-PS Converter2/RConn1
  Electrical Reference2/LConn1 -- Switch/RConn2
  Electrical Reference1/LConn1 -- Resistor1/RConn1
  Variable Inductor/RConn1 -- Variable Resistor/LConn2
  Simulink-PS Converter3/RConn1 -- Variable Inductor/LConn1
  Simulink-PS Converter4/RConn1 -- Variable Resistor/LConn1

== system InductionHeating_bb_4/InitializationBlock ==

== system InductionHeating_bb_4/MATE_Equivalent ==
